simulink model "drone_position_control_sta_z_tuned"  (R2022a)
settings: Solver=ode4  StartTime=0.0  StopTime=42  FixedStep=.001  RelTol=1e-3
model workspace (MAT data in the model file):
  AttDyna_Ixx = 0.0211
  AttDyna_Iyy = 0.0219
  AttDyna_Izz = 0.0366
  AttDyna_JRP = 0.0001287
  ConEfficiency_drone_R = 0.225
  ConEfficiency_drone_cM = 1.779e-07
  ConEfficiency_drone_cT = 1.105e-05
  HeightNominalPlant = [1.4 9.8 1.105e-05 1148 -141.4]
  HeightSTAParams = [20 12 0.01 -22 8 8 0.005 3 5]
  PosDyna_GravityAcc = 9.8
  PosDyna_Mass = 1.4
  PowerUnit_CR = 1148
  PowerUnit_Tm = 0.02
  PowerUnit_wb = -141.4
undefined symbols (not defined in the file): earthRadius, Receive, Send
libraries: aerolibfltsims x3, slpidlib x3, aerolibanimutils x1
Description:
  | 高度专用离散 STA：加速度形式、限速前馈、倾斜重力补偿、条件积分。电机 PWM 共用 1000–2000 限幅。标称参数与实际物理参数分开。
settings Model: Creator=ZhangZheng  LastModifiedBy=13501
settings SolverCC: AlgebraicLoopSolver=TrustRegion
settings DataIOCC: ReturnWorkspaceOutputs=off
settings DebuggingCC: UnconnectedInputMsg=warning  UnconnectedOutputMsg=warning  UnconnectedLineMsg=warning  SFMachineParentedDataDiag=warning  ArithmeticOperatorsInVariantConditions=warning
settings SFSimCC: SimUseLocalCustomCode=off  CustomCodeUndefinedFunction=UseInterfaceOnly
settings RTWCC: RTWUseLocalCustomCode=off

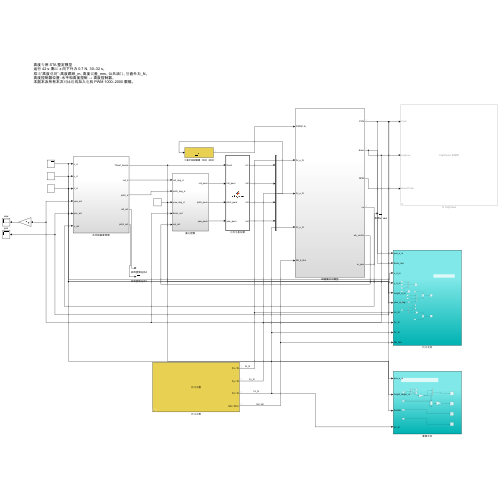
[thumbnail: Simulink's stored preview of the top-level diagram]
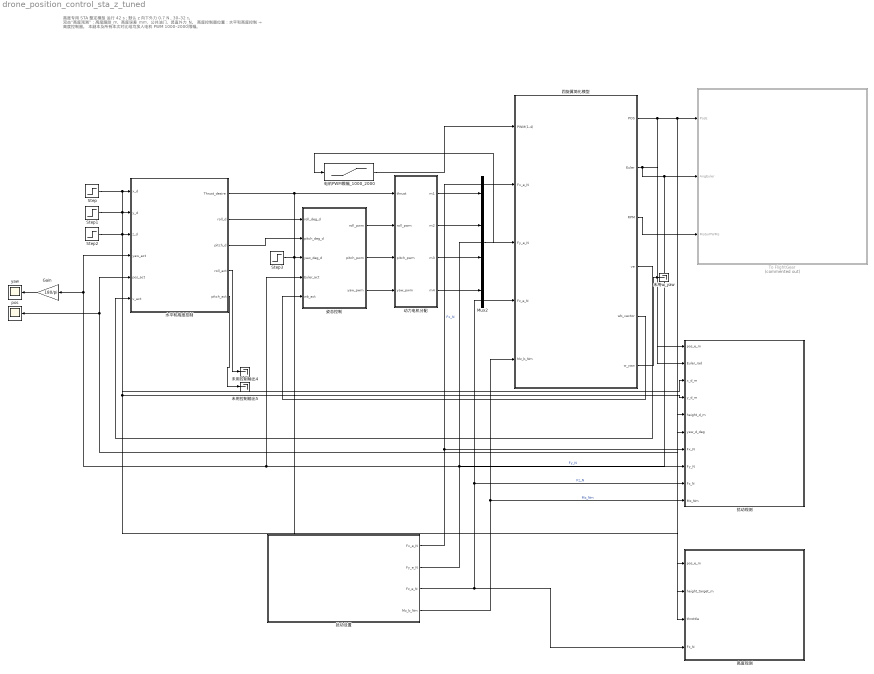
== system drone_position_control_sta_z_tuned ==
  note: 高度专用 STA 整定模型
      | 运行 42 s；默认 z 向下外力 0.7 N，30–32 s。
      | 双击“高度观测”：高度跟踪_m、高度误差_mm、公共油门、竖直外力_N。
      | 高度控制器位置：水平和高度控制 → 高度控制器。
      | 本副本及所有本次对比组均加入电机 PWM 1000–2000 限幅。
  Gain : Gain  Gain=180/pi
  Mux2 : Mux
  Step : Step  Time=5  After=5  SampleTime=0
  Step1 : Step  Time=10  After=5  SampleTime=0
  Step2 : Step  Time=0  After=10  SampleTime=0
  Step3 : Step  Time=15  After=5  SampleTime=0
  To FlightGear : Subsystem  Commented=on
      mask Display: disp('FlightGear 未启用')
  pos : Scope
  yaw : Scope
  动力电机分配 : MATLAB Function  TreatAsAtomicUnit=on
  四旋翼简化模型 : Subsystem
  姿态控制 : Subsystem
  扰动观测 : Subsystem
  扰动设置 : Subsystem  mask{Fx=0, Fy=0, Fz=0.7, Mz=0, t_on=30, t_off=32}
      mask prompts: Fx "x 向外力 Fx (N)"; Fy "y 向外力 Fy (N)"; Fz "z 向外力 Fz (N，向下为正)"; Mz "偏航力矩 Mz (N*m，绕机体 z 轴)"; t_on "施加时刻 (s)"; t_off "撤去时刻 (s)"
      mask help:
      | 默认：x 方向 0.7 N，30–32 s。其余通道为 0。
      | 单轴比较时只开启一个分量。y / z 测试使用 0.7 N，yaw 使用 0.02 N*m。
      | Fx、Fy、Fz 在惯性系表达；Mz 沿机体 z 轴。施加区间为 [施加时刻, 撤去时刻)。
      mask init:
      | validateattributes([Fx Fy Fz Mz],{'double'},{'real','finite','vector','numel',4});
      | validateattributes(t_on,{'double'},{'real','finite','scalar','nonnegative'});
      | validateattributes(t_off,{'double'},{'real','finite','scalar','>',t_on});
      mask Display:
      | disp('扰动设置');
      | port_label('output',1,'Fx / N');
      | port_label('output',2,'Fy / N');
      | port_label('output',3,'Fz / N');
      | port_label('output',4,'Mz / N*m');
  未用w_yaw : Terminator
  未用控制输出4 : Terminator
  未用控制输出5 : Terminator
  水平和高度控制 : Subsystem
  电机PWM限幅_1000_2000 : Saturate  UpperLimit=2000  LowerLimit=1000
  高度观测 : Subsystem
  wires:
  动力电机分配/4(m4) -> Mux2/4
  动力电机分配/3(m3) -> Mux2/3
  动力电机分配/2(m2) -> Mux2/2
  动力电机分配/1(m1) -> Mux2/1
  四旋翼简化模型/1(POS) -> 水平和高度控制/5(pos_act), pos/1, To FlightGear/1(PosE), 高度观测/1(pos_e_m), 扰动观测/1(pos_e_m)
  四旋翼简化模型/3(RPM) -> To FlightGear/3(MotorPWMs)
  姿态控制/1(roll_pwm) -> 动力电机分配/2(roll_pwm)
  姿态控制/2(pitch_pwm) -> 动力电机分配/3(pitch_pwm)
  姿态控制/3(yaw_pwm) -> 动力电机分配/4(yaw_pwm)
  四旋翼简化模型/5(wb_vector) -> 姿态控制/5(wb_act)
  四旋翼简化模型/2(Euler) -> 水平和高度控制/4(yaw_act), Gain/1, 姿态控制/4(Euler_act), To FlightGear/2(AngEuler), 扰动观测/2(Euler_rad)
  四旋翼简化模型/4(ve) -> 水平和高度控制/6(v_act)
  水平和高度控制/1(Thrust_desire) -> 动力电机分配/1(thrust), 高度观测/3(throttle)
  水平和高度控制/2(roll_d) -> 姿态控制/1(roll_deg_d)
  水平和高度控制/3(pitch_d) -> 姿态控制/2(pitch_deg_d)
  Step/1 -> 水平和高度控制/1(x_d), 扰动观测/3(x_d_m)
  Step1/1 -> 水平和高度控制/2(y_d), 扰动观测/4(y_d_m)
  Step2/1 -> 扰动观测/5(height_d_m), 高度观测/2(height_target_m), 水平和高度控制/3(z_d)
  Step3/1 -> 姿态控制/3(yaw_deg_d), 扰动观测/6(yaw_d_deg)
  Gain/1 -> yaw/1
  水平和高度控制/4(roll_act) -> 未用控制输出4/1
  水平和高度控制/5(pitch_act) -> 未用控制输出5/1
  四旋翼简化模型/6(w_yaw) -> 未用w_yaw/1
  扰动设置/1(Fx_e_N) -> 四旋翼简化模型/2(Fx_e_N), 扰动观测/7(Fx_N)  "Fx_N"
  扰动设置/2(Fy_e_N) -> 四旋翼简化模型/3(Fy_e_N), 扰动观测/8(Fy_N)  "Fy_N"
  扰动设置/3(Fz_e_N) -> 四旋翼简化模型/4(Fz_e_N), 扰动观测/9(Fz_N), 高度观测/4(Fz_N)  "Fz_N"
  扰动设置/4(Mz_b_Nm) -> 四旋翼简化模型/5(Mz_b_Nm), 扰动观测/10(Mz_Nm)  "Mz_Nm"
  Mux2/1 -> 电机PWM限幅_1000_2000/1
  电机PWM限幅_1000_2000/1 -> 四旋翼简化模型/1(PWM(1-4))

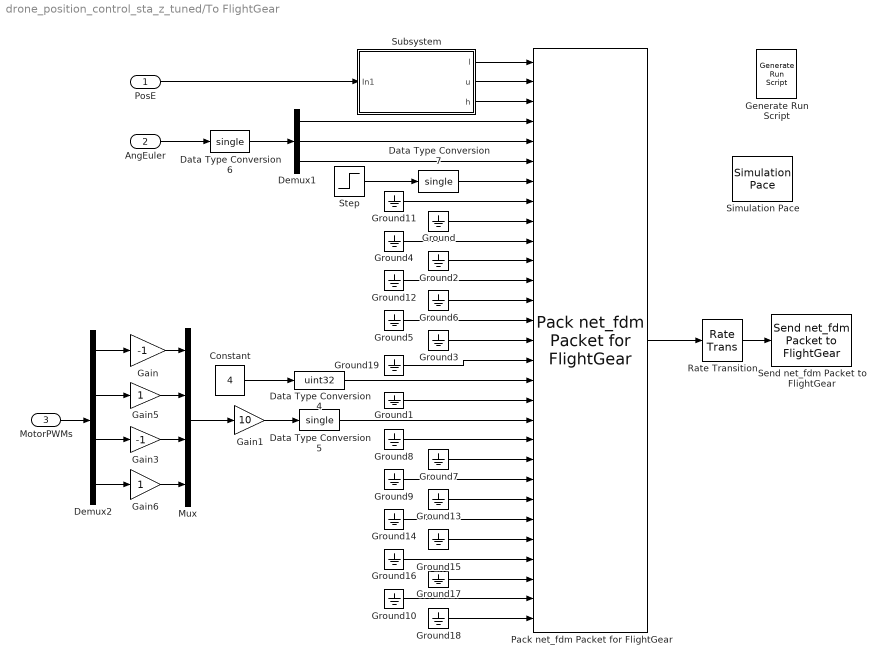
== system drone_position_control_sta_z_tuned/To FlightGear ==
  PosE : Inport
  AngEuler : Inport  Port=2
  MotorPWMs : Inport  Port=3
  Constant : Constant  Value=4
  Data Type Conversion4 : DataTypeConversion  OutDataTypeStr=uint32  SaturateOnIntegerOverflow=off  RndMeth=Floor
  Data Type Conversion5 : DataTypeConversion  OutDataTypeStr=single  SaturateOnIntegerOverflow=off  RndMeth=Floor
  Data Type Conversion6 : DataTypeConversion  OutDataTypeStr=single  SaturateOnIntegerOverflow=off  RndMeth=Floor
  Data Type Conversion7 : DataTypeConversion  OutDataTypeStr=single  SaturateOnIntegerOverflow=off  RndMeth=Floor
  Demux1 : Demux  Outputs=3
  Demux2 : Demux
  Gain : Gain  Gain=-1
  Gain1 : Gain  Gain=10
  Gain3 : Gain  Gain=-1
  Gain5 : Gain
  Gain6 : Gain
  Generate Run Script : aerolibfltsims/Generate Run Script  Architecture=Win64  dataFlow=Send-Receive  GeometryModelName=myownUAV  AirportId=KSFO  RunwayId=0  InitialAltitude=0  InitialHeading=0  OffsetDistance=0  OffsetAzimuth=0  InstallScenery=off  DisableShaders=off  OriginAddress=127.0.0.1  DestinationPort=5502  OriginPort=5505  LocalAddress=127.0.0.1  OutputFileName=runfg.bat  FlightGearBaseDirectory=E:\PX4PSP\FlightGear 2016.1.2
  Ground{,1..19} (20 alike) : Ground
  Mux : Mux
  Pack net_fdm Packet for FlightGear : aerolibfltsims/Pack net_fdm Packet for FlightGear  FlightGearVersion=v2016.1  ShowPositionAttitudeInputs=on  ShowVelocityAccelerationInputs=off  ShowControlSurfacePositionInputs=on  ShowEngineFuelInputs=on  ShowLandingGearInputs=off  ShowEnvironmentInputs=off  SampleTime=0.01  packetVersion=24
      settings: SourceProductBaseCode=AE
  Rate Transition : RateTransition
  Send net_fdm Packet to FlightGear : aerolibfltsims/Send net_fdm Packet to FlightGear  DestinationIpAddress=127.0.0.1  DestinationPort=5502  LocalIpPort=-1  varLen=off  SampleTime=0.005
      settings: SourceProductBaseCode=AE
  Simulation Pace : aerolibanimutils/Simulation Pace  SimulationPace=1  SleepMode=MATLAB Thread  OutputPaceError=off  SampleTime=-1
      settings: AttributesFormatString=%<SimulationPace> sec/sec
  Step : Step  Time=5  SampleTime=0
  Subsystem : Subsystem
  wires:
  Pack net_fdm Packet for FlightGear/1 -> Rate Transition/1
  Data Type Conversion7/1 -> Pack net_fdm Packet for FlightGear/7
  Ground8/1 -> Pack net_fdm Packet for FlightGear/20
  Ground/1 -> Pack net_fdm Packet for FlightGear/9
  Ground7/1 -> Pack net_fdm Packet for FlightGear/21
  Ground9/1 -> Pack net_fdm Packet for FlightGear/22
  Ground13/1 -> Pack net_fdm Packet for FlightGear/23
  Ground14/1 -> Pack net_fdm Packet for FlightGear/24
  Ground15/1 -> Pack net_fdm Packet for FlightGear/25
  Ground16/1 -> Pack net_fdm Packet for FlightGear/26
  Ground17/1 -> Pack net_fdm Packet for FlightGear/27
  Ground10/1 -> Pack net_fdm Packet for FlightGear/28
  Ground18/1 -> Pack net_fdm Packet for FlightGear/29
  Step/1 -> Data Type Conversion7/1
  Data Type Conversion4/1 -> Pack net_fdm Packet for FlightGear/17
  Ground1/1 -> Pack net_fdm Packet for FlightGear/18
  Ground3/1 -> Pack net_fdm Packet for FlightGear/15
  Ground5/1 -> Pack net_fdm Packet for FlightGear/14
  Ground6/1 -> Pack net_fdm Packet for FlightGear/13
  Ground4/1 -> Pack net_fdm Packet for FlightGear/10
  Ground11/1 -> Pack net_fdm Packet for FlightGear/8
  Constant/1 -> Data Type Conversion4/1
  Data Type Conversion5/1 -> Pack net_fdm Packet for FlightGear/19
  Ground2/1 -> Pack net_fdm Packet for FlightGear/11
  Ground12/1 -> Pack net_fdm Packet for FlightGear/12
  AngEuler/1 -> Data Type Conversion6/1
  MotorPWMs/1 -> Demux2/1
  Mux/1 -> Gain1/1
  Demux2/1 -> Gain/1
  Demux2/3 -> Gain3/1
  Gain/1 -> Mux/1
  Gain3/1 -> Mux/3
  Demux2/2 -> Gain5/1
  Gain5/1 -> Mux/2
  Demux2/4 -> Gain6/1
  Gain6/1 -> Mux/4
  Rate Transition/1 -> Send net_fdm Packet to FlightGear/1
  PosE/1 -> Subsystem/1(In1)
  Subsystem/1("l ") -> Pack net_fdm Packet for FlightGear/1
  Subsystem/2(u) -> Pack net_fdm Packet for FlightGear/2
  Subsystem/3(h) -> Pack net_fdm Packet for FlightGear/3
  Ground19/1 -> Pack net_fdm Packet for FlightGear/16
  Demux1/1 -> Pack net_fdm Packet for FlightGear/4
  Demux1/2 -> Pack net_fdm Packet for FlightGear/5
  Demux1/3 -> Pack net_fdm Packet for FlightGear/6
  Data Type Conversion6/1 -> Demux1/1
  Gain1/1 -> Data Type Conversion5/1

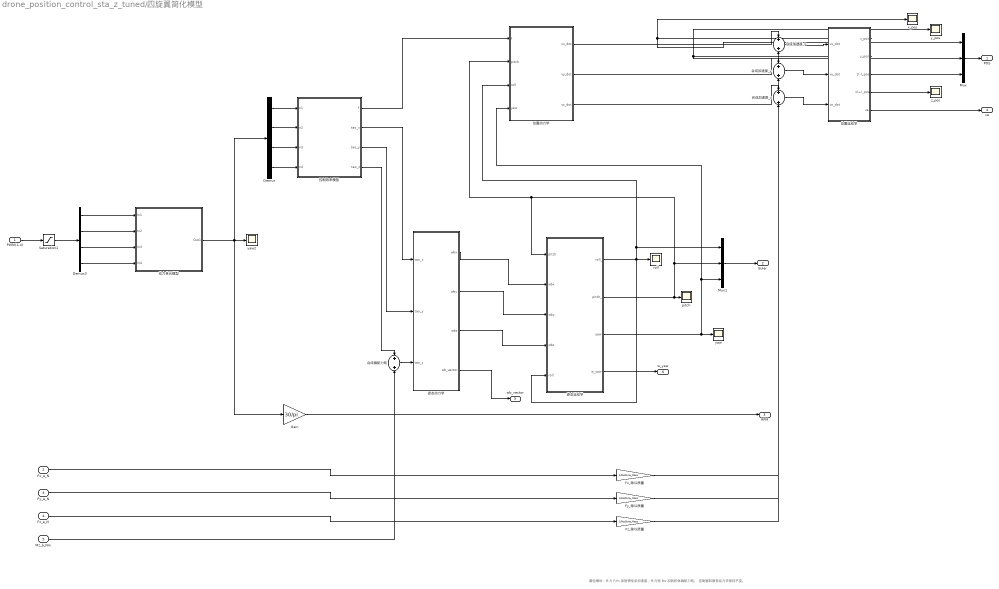
== system drone_position_control_sta_z_tuned/四旋翼简化模型 ==
  note: 黄色模块：外力 F/m 加到惯性系加速度；外力矩 Mz 加到机体偏航力矩。
      | 控制器和原有动力学保持不变。
  PWM(1-4) : Inport
  Fx_e_N : Inport  Port=2
  Fy_e_N : Inport  Port=3
  Fz_e_N : Inport  Port=4
  Mz_b_Nm : Inport  Port=5
  Demux : Demux
  Demux3 : Demux
  Fx_除以质量 : Gain  Gain=1/PosDyna_Mass
  Fy_除以质量 : Gain  Gain=1/PosDyna_Mass
  Fz_除以质量 : Gain  Gain=1/PosDyna_Mass
  Gain : Gain  Gain=30/pi
  Mux : Mux  Inputs=3
  Mux1 : Mux  Inputs=3
  Saturation1 : Saturate  UpperLimit=2000  LowerLimit=1000
  pitch : Scope
  roll : Scope
  x_pos : Scope
  y_pos : Scope
  yaw : Scope
  yaw2 : Scope
  z_pos : Scope
  位置动力学 : Subsystem
  位置运动学 : Subsystem
  动力单元模型 : Subsystem
  合成偏航力矩 : Sum
  合成加速度_x : Sum
  合成加速度_y : Sum
  合成加速度_z : Sum
  姿态动力学 : Subsystem
  姿态运动学 : Subsystem
  控制效率模型 : Subsystem
  POS : Outport  VectorParamsAs1DForOutWhenUnconnected=off
  Euler : Outport  Port=2  VectorParamsAs1DForOutWhenUnconnected=off
  RPM : Outport  Port=3  VectorParamsAs1DForOutWhenUnconnected=off
  ve : Outport  Port=4  VectorParamsAs1DForOutWhenUnconnected=off
  wb_vector : Outport  Port=5  VectorParamsAs1DForOutWhenUnconnected=off
  w_yaw : Outport  Port=6  VectorParamsAs1DForOutWhenUnconnected=off
  wires:
  Saturation1/1 -> Demux3/1
  姿态运动学/2(pitch_) -> 姿态运动学/1(pitch), 位置动力学/2(pitch), Mux1/2, pitch/1
  Demux/3 -> 控制效率模型/3(n3)
  PWM(1-4)/1 -> Saturation1/1
  Demux3/1 -> 动力单元模型/1(In1)
  Gain/1 -> RPM/1
  控制效率模型/3(tao_y) -> 姿态动力学/2(tao_y)
  Demux3/3 -> 动力单元模型/3(In3)
  Mux/1 -> POS/1
  Demux3/2 -> 动力单元模型/2(In2)
  Demux/2 -> 控制效率模型/2(n2)
  动力单元模型/1(Out1) -> Demux/1, yaw2/1, Gain/1
  Demux3/4 -> 动力单元模型/4(In4)
  Mux1/1 -> Euler/1
  控制效率模型/1(f) -> 位置动力学/1(f)
  Demux/4 -> 控制效率模型/4(n4)
  Demux/1 -> 控制效率模型/1(n1)
  控制效率模型/2(tao_x) -> 姿态动力学/1(tao_x)
  姿态动力学/1(wbx) -> 姿态运动学/2(wbx)
  姿态运动学/1(roll_) -> 姿态运动学/5(roll), roll/1, 位置动力学/3(roll), Mux1/1
  姿态动力学/4(wb_vector) -> wb_vector/1
  姿态运动学/3(yaw) -> 位置动力学/4(yaw), Mux1/3, yaw/1
  姿态动力学/3(wbz) -> 姿态运动学/4(wbz)
  姿态动力学/2(wby) -> 姿态运动学/3(wby)
  姿态运动学/4(w_yaw) -> w_yaw/1
  位置运动学/1(x_pos) -> x_pos/1, Mux/1
  位置运动学/2(y_pos) -> Mux/2, y_pos/1
  位置运动学/3(z(-)_pos) -> Mux/3
  位置运动学/4(z(+)_pos) -> z_pos/1
  位置运动学/5(ve) -> ve/1
  Fx_e_N/1 -> Fx_除以质量/1
  位置动力学/1(vx_dot) -> 合成加速度_x/1
  Fx_除以质量/1 -> 合成加速度_x/2
  合成加速度_x/1 -> 位置运动学/1(vx_dot)
  Fy_e_N/1 -> Fy_除以质量/1
  位置动力学/2(vy_dot) -> 合成加速度_y/1
  Fy_除以质量/1 -> 合成加速度_y/2
  合成加速度_y/1 -> 位置运动学/2(vy_dot)
  Fz_e_N/1 -> Fz_除以质量/1
  位置动力学/3(vz_dot) -> 合成加速度_z/1
  Fz_除以质量/1 -> 合成加速度_z/2
  合成加速度_z/1 -> 位置运动学/3(vz_dot)
  控制效率模型/4(tao_z) -> 合成偏航力矩/1
  Mz_b_Nm/1 -> 合成偏航力矩/2
  合成偏航力矩/1 -> 姿态动力学/3(tao_z)

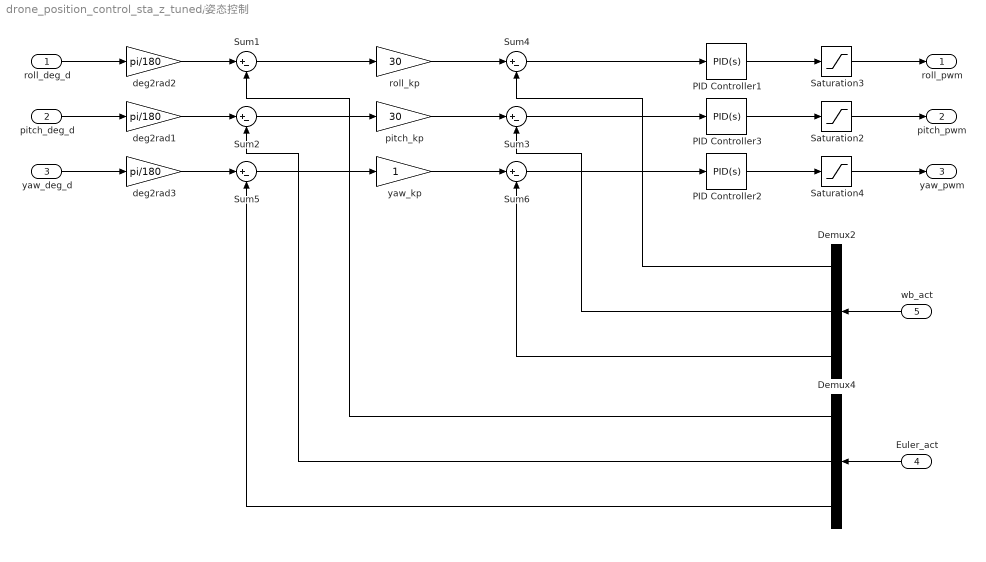
== system drone_position_control_sta_z_tuned/姿态控制 ==
  roll_deg_d : Inport
  pitch_deg_d : Inport  Port=2
  yaw_deg_d : Inport  Port=3
  Euler_act : Inport  Port=4
  wb_act : Inport  Port=5
  Demux2 : Demux  Outputs=3
  Demux4 : Demux  Outputs=3
  PID Controller1 : slpidlib/PID Controller  Controller=PID  Form=Parallel  TimeDomain=Continuous-time  UseExternalTs=off  SampleTime=-1  IntegratorMethod=Forward Euler  FilterMethod=Forward Euler  ControllerParametersSource=internal  P=0.3  I=1.4  UseKiTs=off  D=0.01  N=100  UseFilter=on  TunerSelectOption=Transfer Function Based (PID Tuner App)  InitialConditionSource=internal  InitialConditionForIntegrator=0  InitialConditionForFilter=0  DifferentiatorICPrevScaledInput=0  ExternalReset=none  TrackingMode=off  Kt=1  LimitOutput=off  SatLimitsSource=internal  UpperSaturationLimit=inf  LowerSaturationLimit=-inf  LinearizeAsGain=on  AntiWindupMode=none  Kb=1  POutMin=[]  POutMax=[]  IOutMin=[]  IOutMax=[]  DOutMin=[]  DOutMax=[]  NOutMin=[]  NOutMax=[]  SumOutMin=[]  SumOutMax=[]  SaturationOutMin=[]  SaturationOutMax=[]  PParamMin=[]  PParamMax=[]  IParamMin=[]  IParamMax=[]  DParamMin=[]  DParamMax=[]  NParamMin=[]  NParamMax=[]  KbParamMin=[]  KbParamMax=[]  KtParamMin=[]  KtParamMax=[]  KbOutMin=[]  KbOutMax=[]  KtOutMin=[]  KtOutMax=[]  IntegratorOutMin=[]  IntegratorOutMax=[]  FilterOutMin=[]  FilterOutMax=[]  SumI1OutMin=[]  SumI1OutMax=[]  SumI2OutMin=[]  SumI2OutMax=[]  SumI3OutMin=[]  SumI3OutMax=[]  SumI4OutMin=[]  SumI4OutMax=[]  SumDOutMin=[]  SumDOutMax=[]  DifferentiatorOutMin=[]  DifferentiatorOutMax=[]  FilterDiffOutCoefMin=[]  FilterDiffOutCoefMax=[]  ReciprocalOutMin=[]  ReciprocalOutMax=[]  SumDenOutMin=[]  SumDenOutMax=[]  SumNumOutMin=[]  SumNumOutMax=[]  DivideOutMin=[]  DivideOutMax=[]  UdiffTsProdOutMin=[]  UdiffTsProdOutMax=[]  NTsProdOutMin=[]  NTsProdOutMax=[]  UintegralTsProdOutMin=[]  UintegralTsProdOutMax=[]  UngainTsProdOutMin=[]  UngainTsProdOutMax=[]  IntegratorContinuousStateAttributes=''  IntegratorStateMustResolveToSignalObject=off  IntegratorRTWStateStorageClass=Auto  FilterContinuousStateAttributes=''  FilterStateMustResolveToSignalObject=off  FilterRTWStateStorageClass=Auto  ParallelPVariant=InternalParameters  IdealPVariant=Disabled  IVariant=InternalParameters  DVariant=InternalParameters  IntegratorVariant=Continuous  SatVariant=Disabled  AWVariant=Passthrough  PCopyVariant=Disabled  TRVariant=Disabled  FdbkBlocksVariant=Forward  IdealPFdbkVariant=Disabled  SatFdbkVariant=Disabled  DerivativeFilterVariant=ContFilter  NVariant=InternalParameters  NCopyVariant=Disabled  FilterICVariant=InternalICsFilter  IntegratorICVariant=InternalICs  ExternalResetVariant=Disabled  TRSumVariant=Passthrough  SumFdbkVariant=Disabled  SumVariant=Sum_PID  TsampFilterVariant=InternalTs  TsampNgainVariant=Passthrough  TsampIntegralVariant=Passthrough  ExternalSaturationOutDataTypeStr=Inherit: Same as second input  aMode=0
  PID Controller2 : slpidlib/PID Controller  Controller=PID  Form=Parallel  TimeDomain=Continuous-time  UseExternalTs=off  SampleTime=-1  IntegratorMethod=Forward Euler  FilterMethod=Forward Euler  ControllerParametersSource=internal  P=20  I=0  UseKiTs=off  D=0.1  N=100  UseFilter=on  TunerSelectOption=Transfer Function Based (PID Tuner App)  InitialConditionSource=internal  InitialConditionForIntegrator=0  InitialConditionForFilter=0  DifferentiatorICPrevScaledInput=0  ExternalReset=none  TrackingMode=off  Kt=1  LimitOutput=off  SatLimitsSource=internal  UpperSaturationLimit=inf  LowerSaturationLimit=-inf  LinearizeAsGain=on  AntiWindupMode=none  Kb=1  POutMin=[]  POutMax=[]  IOutMin=[]  IOutMax=[]  DOutMin=[]  DOutMax=[]  NOutMin=[]  NOutMax=[]  SumOutMin=[]  SumOutMax=[]  SaturationOutMin=[]  SaturationOutMax=[]  PParamMin=[]  PParamMax=[]  IParamMin=[]  IParamMax=[]  DParamMin=[]  DParamMax=[]  NParamMin=[]  NParamMax=[]  KbParamMin=[]  KbParamMax=[]  KtParamMin=[]  KtParamMax=[]  KbOutMin=[]  KbOutMax=[]  KtOutMin=[]  KtOutMax=[]  IntegratorOutMin=[]  IntegratorOutMax=[]  FilterOutMin=[]  FilterOutMax=[]  SumI1OutMin=[]  SumI1OutMax=[]  SumI2OutMin=[]  SumI2OutMax=[]  SumI3OutMin=[]  SumI3OutMax=[]  SumI4OutMin=[]  SumI4OutMax=[]  SumDOutMin=[]  SumDOutMax=[]  DifferentiatorOutMin=[]  DifferentiatorOutMax=[]  FilterDiffOutCoefMin=[]  FilterDiffOutCoefMax=[]  ReciprocalOutMin=[]  ReciprocalOutMax=[]  SumDenOutMin=[]  SumDenOutMax=[]  SumNumOutMin=[]  SumNumOutMax=[]  DivideOutMin=[]  DivideOutMax=[]  UdiffTsProdOutMin=[]  UdiffTsProdOutMax=[]  NTsProdOutMin=[]  NTsProdOutMax=[]  UintegralTsProdOutMin=[]  UintegralTsProdOutMax=[]  UngainTsProdOutMin=[]  UngainTsProdOutMax=[]  IntegratorContinuousStateAttributes=''  IntegratorStateMustResolveToSignalObject=off  IntegratorRTWStateStorageClass=Auto  FilterContinuousStateAttributes=''  FilterStateMustResolveToSignalObject=off  FilterRTWStateStorageClass=Auto  ParallelPVariant=InternalParameters  IdealPVariant=Disabled  IVariant=InternalParameters  DVariant=InternalParameters  IntegratorVariant=Continuous  SatVariant=Disabled  AWVariant=Passthrough  PCopyVariant=Disabled  TRVariant=Disabled  FdbkBlocksVariant=Forward  IdealPFdbkVariant=Disabled  SatFdbkVariant=Disabled  DerivativeFilterVariant=ContFilter  NVariant=InternalParameters  NCopyVariant=Disabled  FilterICVariant=InternalICsFilter  IntegratorICVariant=InternalICs  ExternalResetVariant=Disabled  TRSumVariant=Passthrough  SumFdbkVariant=Disabled  SumVariant=Sum_PID  TsampFilterVariant=InternalTs  TsampNgainVariant=Passthrough  TsampIntegralVariant=Passthrough  ExternalSaturationOutDataTypeStr=Inherit: Same as second input  aMode=0
  PID Controller3 : slpidlib/PID Controller  Controller=PID  Form=Parallel  TimeDomain=Continuous-time  UseExternalTs=off  SampleTime=-1  IntegratorMethod=Forward Euler  FilterMethod=Forward Euler  ControllerParametersSource=internal  P=0.3  I=1.4  UseKiTs=off  D=0.01  N=100  UseFilter=on  TunerSelectOption=Transfer Function Based (PID Tuner App)  InitialConditionSource=internal  InitialConditionForIntegrator=0  InitialConditionForFilter=0  DifferentiatorICPrevScaledInput=0  ExternalReset=none  TrackingMode=off  Kt=1  LimitOutput=off  SatLimitsSource=internal  UpperSaturationLimit=inf  LowerSaturationLimit=-inf  LinearizeAsGain=on  AntiWindupMode=none  Kb=1  POutMin=[]  POutMax=[]  IOutMin=[]  IOutMax=[]  DOutMin=[]  DOutMax=[]  NOutMin=[]  NOutMax=[]  SumOutMin=[]  SumOutMax=[]  SaturationOutMin=[]  SaturationOutMax=[]  PParamMin=[]  PParamMax=[]  IParamMin=[]  IParamMax=[]  DParamMin=[]  DParamMax=[]  NParamMin=[]  NParamMax=[]  KbParamMin=[]  KbParamMax=[]  KtParamMin=[]  KtParamMax=[]  KbOutMin=[]  KbOutMax=[]  KtOutMin=[]  KtOutMax=[]  IntegratorOutMin=[]  IntegratorOutMax=[]  FilterOutMin=[]  FilterOutMax=[]  SumI1OutMin=[]  SumI1OutMax=[]  SumI2OutMin=[]  SumI2OutMax=[]  SumI3OutMin=[]  SumI3OutMax=[]  SumI4OutMin=[]  SumI4OutMax=[]  SumDOutMin=[]  SumDOutMax=[]  DifferentiatorOutMin=[]  DifferentiatorOutMax=[]  FilterDiffOutCoefMin=[]  FilterDiffOutCoefMax=[]  ReciprocalOutMin=[]  ReciprocalOutMax=[]  SumDenOutMin=[]  SumDenOutMax=[]  SumNumOutMin=[]  SumNumOutMax=[]  DivideOutMin=[]  DivideOutMax=[]  UdiffTsProdOutMin=[]  UdiffTsProdOutMax=[]  NTsProdOutMin=[]  NTsProdOutMax=[]  UintegralTsProdOutMin=[]  UintegralTsProdOutMax=[]  UngainTsProdOutMin=[]  UngainTsProdOutMax=[]  IntegratorContinuousStateAttributes=''  IntegratorStateMustResolveToSignalObject=off  IntegratorRTWStateStorageClass=Auto  FilterContinuousStateAttributes=''  FilterStateMustResolveToSignalObject=off  FilterRTWStateStorageClass=Auto  ParallelPVariant=InternalParameters  IdealPVariant=Disabled  IVariant=InternalParameters  DVariant=InternalParameters  IntegratorVariant=Continuous  SatVariant=Disabled  AWVariant=Passthrough  PCopyVariant=Disabled  TRVariant=Disabled  FdbkBlocksVariant=Forward  IdealPFdbkVariant=Disabled  SatFdbkVariant=Disabled  DerivativeFilterVariant=ContFilter  NVariant=InternalParameters  NCopyVariant=Disabled  FilterICVariant=InternalICsFilter  IntegratorICVariant=InternalICs  ExternalResetVariant=Disabled  TRSumVariant=Passthrough  SumFdbkVariant=Disabled  SumVariant=Sum_PID  TsampFilterVariant=InternalTs  TsampNgainVariant=Passthrough  TsampIntegralVariant=Passthrough  ExternalSaturationOutDataTypeStr=Inherit: Same as second input  aMode=0
  Saturation2 : Saturate  UpperLimit=1  LowerLimit=-1
  Saturation3 : Saturate  UpperLimit=1  LowerLimit=-1
  Saturation4 : Saturate  UpperLimit=1  LowerLimit=-1
  Sum{1..6} (6 alike) : Sum  Inputs=|+-
  deg2rad1 : Gain  Gain=pi/180
  deg2rad2 : Gain  Gain=pi/180
  deg2rad3 : Gain  Gain=pi/180
  pitch_kp : Gain  Gain=30
  roll_kp : Gain  Gain=30
  yaw_kp : Gain
  roll_pwm : Outport  VectorParamsAs1DForOutWhenUnconnected=off
  pitch_pwm : Outport  Port=2  VectorParamsAs1DForOutWhenUnconnected=off
  yaw_pwm : Outport  Port=3  VectorParamsAs1DForOutWhenUnconnected=off
  wires:
  PID Controller1/1 -> Saturation3/1
  roll_deg_d/1 -> deg2rad2/1
  pitch_deg_d/1 -> deg2rad1/1
  Saturation2/1 -> pitch_pwm/1
  Sum2/1 -> pitch_kp/1
  Saturation3/1 -> roll_pwm/1
  PID Controller3/1 -> Saturation2/1
  deg2rad1/1 -> Sum2/1
  Sum1/1 -> roll_kp/1
  roll_kp/1 -> Sum4/1
  Saturation4/1 -> yaw_pwm/1
  yaw_kp/1 -> Sum6/1
  pitch_kp/1 -> Sum3/1
  deg2rad2/1 -> Sum1/1
  wb_act/1 -> Demux2/1
  PID Controller2/1 -> Saturation4/1
  yaw_deg_d/1 -> deg2rad3/1
  Demux2/3 -> Sum6/2
  deg2rad3/1 -> Sum5/1
  Demux2/2 -> Sum3/2
  Sum5/1 -> yaw_kp/1
  Demux4/3 -> Sum5/2
  Demux2/1 -> Sum4/2
  Demux4/2 -> Sum2/2
  Demux4/1 -> Sum1/2
  Euler_act/1 -> Demux4/1
  Sum4/1 -> PID Controller1/1
  Sum3/1 -> PID Controller3/1
  Sum6/1 -> PID Controller2/1

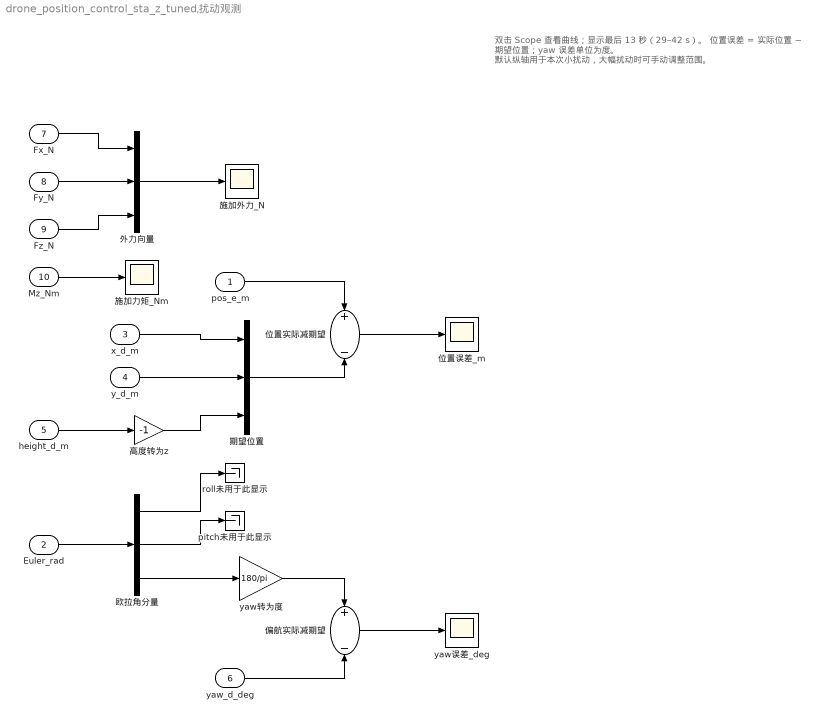
== system drone_position_control_sta_z_tuned/扰动观测 ==
  note: 双击 Scope 查看曲线；显示最后 13 秒（29–42 s）。
      | 位置误差 = 实际位置 − 期望位置；yaw 误差单位为度。
      | 默认纵轴用于本次小扰动，大幅扰动时可手动调整范围。
  pos_e_m : Inport
  Euler_rad : Inport  Port=2
  x_d_m : Inport  Port=3
  y_d_m : Inport  Port=4
  height_d_m : Inport  Port=5
  yaw_d_deg : Inport  Port=6
  Fx_N : Inport  Port=7
  Fy_N : Inport  Port=8
  Fz_N : Inport  Port=9
  Mz_Nm : Inport  Port=10
  pitch未用于此显示 : Terminator
  roll未用于此显示 : Terminator
  yaw误差_deg : Scope
  yaw转为度 : Gain  Gain=180/pi
  位置实际减期望 : Sum  Inputs=+-
  位置误差_m : Scope
  偏航实际减期望 : Sum  Inputs=+-
  外力向量 : Mux  Inputs=3
  施加力矩_Nm : Scope
  施加外力_N : Scope
  期望位置 : Mux  Inputs=3
  欧拉角分量 : Demux  Outputs=3
  高度转为z : Gain  Gain=-1
  wires:
  Mz_Nm/1 -> 施加力矩_Nm/1
  位置实际减期望/1 -> 位置误差_m/1
  高度转为z/1 -> 期望位置/3
  欧拉角分量/3 -> yaw转为度/1
  偏航实际减期望/1 -> yaw误差_deg/1
  外力向量/1 -> 施加外力_N/1
  Fx_N/1 -> 外力向量/1
  Fz_N/1 -> 外力向量/3
  yaw_d_deg/1 -> 偏航实际减期望/2
  Fy_N/1 -> 外力向量/2
  yaw转为度/1 -> 偏航实际减期望/1
  欧拉角分量/2 -> pitch未用于此显示/1
  欧拉角分量/1 -> roll未用于此显示/1
  Euler_rad/1 -> 欧拉角分量/1
  期望位置/1 -> 位置实际减期望/2
  pos_e_m/1 -> 位置实际减期望/1
  height_d_m/1 -> 高度转为z/1
  y_d_m/1 -> 期望位置/2
  x_d_m/1 -> 期望位置/1

== system drone_position_control_sta_z_tuned/扰动设置 ==
  Fx : Gain  Gain=Fx
  Fy : Gain  Gain=Fy
  Fz : Gain  Gain=Fz
  Mz : Gain  Gain=Mz
  持续时间窗口 : Sum
  撤去 : Step  Time=t_off  After=-1  SampleTime=0
  施加 : Step  Time=t_on  SampleTime=0
  Fx_e_N : Outport
  Fy_e_N : Outport  Port=2
  Fz_e_N : Outport  Port=3
  Mz_b_Nm : Outport  Port=4
  wires:
  施加/1 -> 持续时间窗口/1
  撤去/1 -> 持续时间窗口/2
  持续时间窗口/1 -> Fx/1, Fy/1, Fz/1, Mz/1
  Fx/1 -> Fx_e_N/1
  Fy/1 -> Fy_e_N/1
  Fz/1 -> Fz_e_N/1
  Mz/1 -> Mz_b_Nm/1

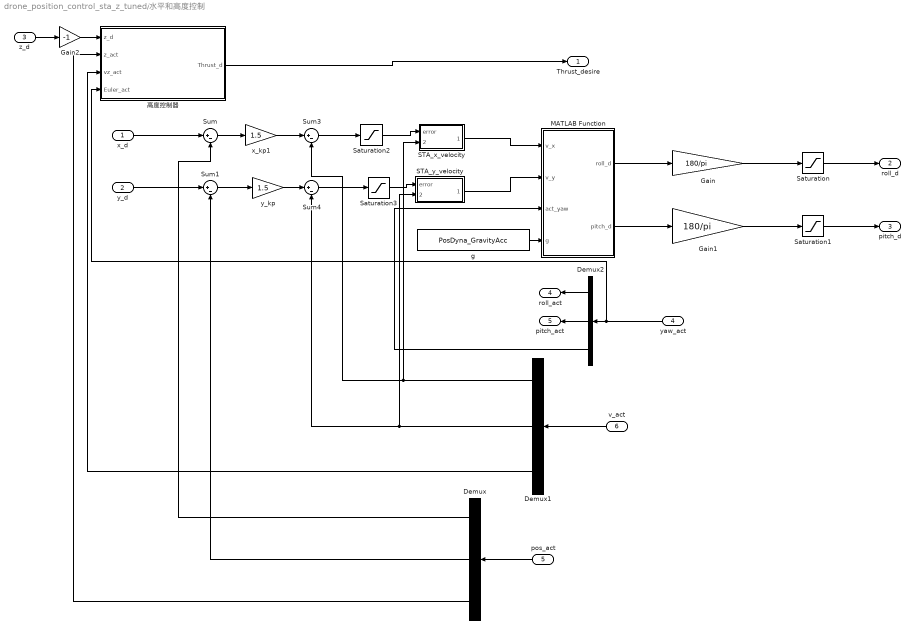
== system drone_position_control_sta_z_tuned/水平和高度控制 ==
  x_d : Inport
  y_d : Inport  Port=2
  z_d : Inport  Port=3
  yaw_act : Inport  Port=4
  pos_act : Inport  Port=5
  v_act : Inport  Port=6
  Demux : Demux  Outputs=3
  Demux1 : Demux  Outputs=3
  Demux2 : Demux  Outputs=3
  Gain : Gain  Gain=180/pi
  Gain1 : Gain  Gain=180/pi
  Gain2 : Gain  Gain=-1
  MATLAB Function : MATLAB Function  TreatAsAtomicUnit=on
  STA_x_velocity : Subsystem  Tag=STA:x_velocity  Description=水平 STA 试验：速度前馈 -lambda*v_actual；条件积分抗饱和；Ts=0.005s。源码 sta_velocity_ff_conditional.m 为说明副本，仿真运行模型内嵌函数。
  STA_y_velocity : Subsystem  Tag=STA:y_velocity  Description=水平 STA 试验：速度前馈 -lambda*v_actual；条件积分抗饱和；Ts=0.005s。源码 sta_velocity_ff_conditional.m 为说明副本，仿真运行模型内嵌函数。
  Saturation : Saturate  UpperLimit=10  LowerLimit=-20
  Saturation1 : Saturate  UpperLimit=10  LowerLimit=-10
  Saturation2 : Saturate  Description=保留完整速度误差；加速度指令在 STA 函数内限幅至正负 1.7 m/s^2。  UpperLimit=inf  LowerLimit=-inf
  Saturation3 : Saturate  Description=保留完整速度误差；加速度指令在 STA 函数内限幅至正负 1.7 m/s^2。  UpperLimit=inf  LowerLimit=-inf
  Sum{,1,3..4} (4 alike) : Sum  Inputs=|+-
  g : Constant  Value=PosDyna_GravityAcc
  x_kp1 : Gain  Gain=1.5
  y_kp : Gain  Gain=1.5
  高度控制器 : Subsystem  Description=高度专用 STA：NED z 向下，加速度单位控制律、限速前馈、倾斜重力补偿、条件积分。参数在模型工作区 HeightSTAParams。
  Thrust_desire : Outport  VectorParamsAs1DForOutWhenUnconnected=off
  roll_d : Outport  Port=2  VectorParamsAs1DForOutWhenUnconnected=off
  pitch_d : Outport  Port=3  VectorParamsAs1DForOutWhenUnconnected=off
  roll_act : Outport  Port=4  VectorParamsAs1DForOutWhenUnconnected=off
  pitch_act : Outport  Port=5  VectorParamsAs1DForOutWhenUnconnected=off
  wires:
  Saturation2/1 -> STA_x_velocity/1(error)
  Demux2/3 -> MATLAB Function/3(act_yaw)
  Demux2/1 -> roll_act/1
  yaw_act/1 -> Demux2/1, 高度控制器/4(Euler_act)
  Demux2/2 -> pitch_act/1
  pos_act/1 -> Demux/1
  Demux/2 -> Sum1/2
  Sum1/1 -> y_kp/1
  Sum4/1 -> Saturation3/1
  y_kp/1 -> Sum4/1
  y_d/1 -> Sum1/1
  Demux/1 -> Sum/2
  z_d/1 -> Gain2/1
  g/1 -> MATLAB Function/4(g)
  v_act/1 -> Demux1/1
  Saturation/1 -> roll_d/1
  Demux1/1 -> Sum3/2, STA_x_velocity/2(actual_velocity)
  MATLAB Function/2(pitch_d) -> Gain1/1
  Saturation1/1 -> pitch_d/1
  STA_x_velocity/1(control) -> MATLAB Function/1(v_x)
  Gain/1 -> Saturation/1
  MATLAB Function/1(roll_d) -> Gain/1
  Sum3/1 -> Saturation2/1
  STA_y_velocity/1(control) -> MATLAB Function/2(v_y)
  Demux1/2 -> Sum4/2, STA_y_velocity/2(actual_velocity)
  Saturation3/1 -> STA_y_velocity/1(error)
  x_kp1/1 -> Sum3/1
  x_d/1 -> Sum/1
  Gain1/1 -> Saturation1/1
  Sum/1 -> x_kp1/1
  高度控制器/1(Thrust_d) -> Thrust_desire/1
  Gain2/1 -> 高度控制器/1(z_d)
  Demux/3 -> 高度控制器/2(z_act)
  Demux1/3 -> 高度控制器/3(vz_act)

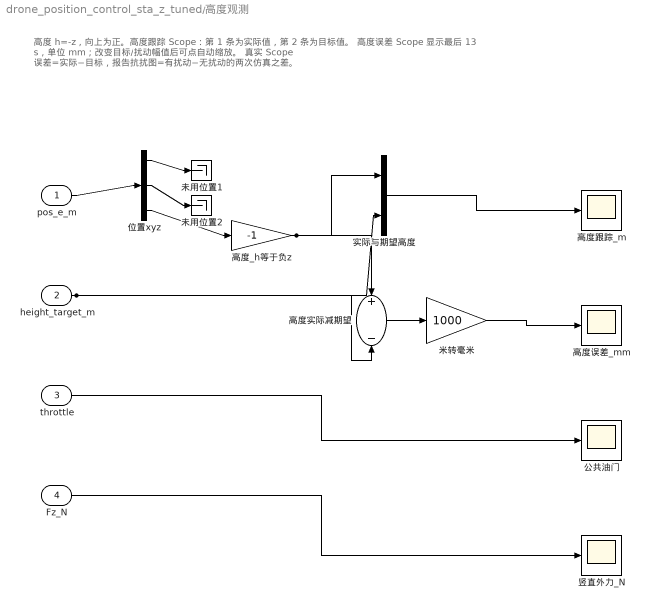
== system drone_position_control_sta_z_tuned/高度观测 ==
  note: 高度 h=-z，向上为正。高度跟踪 Scope：第 1 条为实际值，第 2 条为目标值。
      | 高度误差 Scope 显示最后 13 s，单位 mm；改变目标/扰动幅值后可点自动缩放。
      | 真实 Scope 误差=实际−目标，报告抗扰图=有扰动−无扰动的两次仿真之差。
  pos_e_m : Inport
  height_target_m : Inport  Port=2
  throttle : Inport  Port=3
  Fz_N : Inport  Port=4
  位置xyz : Demux  Outputs=3
  公共油门 : Scope
  实际与期望高度 : Mux  Inputs=2
  未用位置1 : Terminator
  未用位置2 : Terminator
  竖直外力_N : Scope
  米转毫米 : Gain  Gain=1000
  高度_h等于负z : Gain  Gain=-1
  高度实际减期望 : Sum  Inputs=+-
  高度误差_mm : Scope
  高度跟踪_m : Scope
  wires:
  pos_e_m/1 -> 位置xyz/1
  位置xyz/1 -> 未用位置1/1
  位置xyz/2 -> 未用位置2/1
  位置xyz/3 -> 高度_h等于负z/1
  高度_h等于负z/1 -> 实际与期望高度/1, 高度实际减期望/1
  height_target_m/1 -> 实际与期望高度/2, 高度实际减期望/2
  高度实际减期望/1 -> 米转毫米/1
  实际与期望高度/1 -> 高度跟踪_m/1
  米转毫米/1 -> 高度误差_mm/1
  throttle/1 -> 公共油门/1
  Fz_N/1 -> 竖直外力_N/1

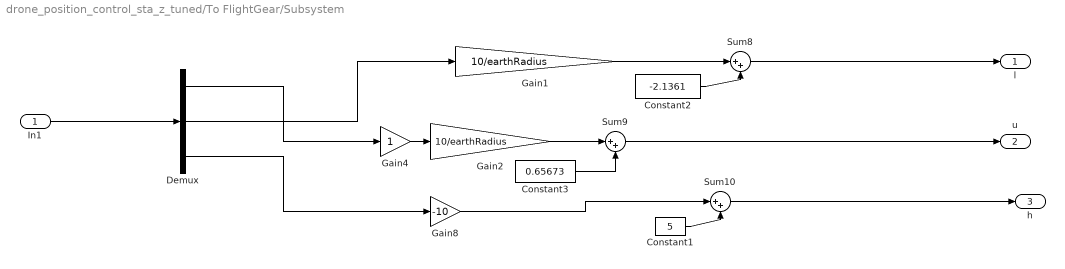
== system drone_position_control_sta_z_tuned/To FlightGear/Subsystem ==
  In1 : Inport
  Constant1 : Constant  Value=5  VectorParams1D=off
  Constant2 : Constant  Value=-2.1361  VectorParams1D=off
  Constant3 : Constant  Value=0.65673  VectorParams1D=off
  Demux : Demux  Outputs=3
  Gain1 : Gain  Gain=10/earthRadius
  Gain2 : Gain  Gain=10/earthRadius
  Gain4 : Gain
  Gain8 : Gain  Gain=-10
  Sum10 : Sum  Inputs=|++
  Sum8 : Sum  Inputs=|++
  Sum9 : Sum  Inputs=|++
  "l " : Outport  VectorParamsAs1DForOutWhenUnconnected=off
  u : Outport  Port=2  VectorParamsAs1DForOutWhenUnconnected=off
  h : Outport  Port=3  VectorParamsAs1DForOutWhenUnconnected=off
  wires:
  Constant3/1 -> Sum9/2
  Constant1/1 -> Sum10/2
  Demux/1 -> Gain4/1
  Demux/3 -> Gain8/1
  Constant2/1 -> Sum8/2
  Gain2/1 -> Sum9/1
  Gain1/1 -> Sum8/1
  Gain8/1 -> Sum10/1
  Demux/2 -> Gain1/1
  Gain4/1 -> Gain2/1
  Sum10/1 -> h/1
  Sum9/1 -> u/1
  In1/1 -> Demux/1
  Sum8/1 -> "l "/1

== system drone_position_control_sta_z_tuned/四旋翼简化模型/位置动力学 ==
  f : Inport
  pitch : Inport  Port=2
  roll : Inport  Port=3
  yaw : Inport  Port=4
  Constant : Constant  Value=PosDyna_Mass
  Constant3 : Constant  Value=PosDyna_GravityAcc
  pos_dyna : MATLAB Function  TreatAsAtomicUnit=on
  vx_dot : Outport  VectorParamsAs1DForOutWhenUnconnected=off
  vy_dot : Outport  Port=2  VectorParamsAs1DForOutWhenUnconnected=off
  vz_dot : Outport  Port=3  VectorParamsAs1DForOutWhenUnconnected=off
  wires:
  pos_dyna/1(vx_dot) -> vx_dot/1
  Constant/1 -> pos_dyna/2(m)
  pos_dyna/3(vz_dot) -> vz_dot/1
  pos_dyna/2(vy_dot) -> vy_dot/1
  Constant3/1 -> pos_dyna/3(g)
  yaw/1 -> pos_dyna/4(yaw)
  pitch/1 -> pos_dyna/5(pitch)
  roll/1 -> pos_dyna/6(roll)
  f/1 -> pos_dyna/1(f)

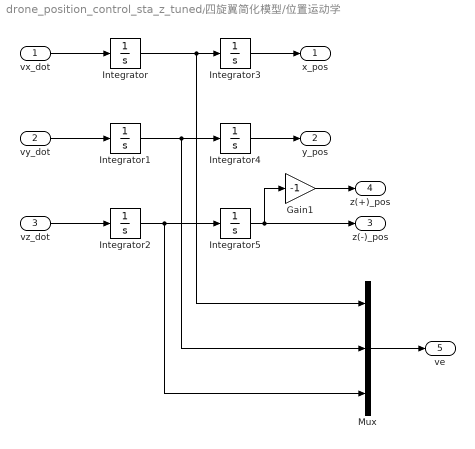
== system drone_position_control_sta_z_tuned/四旋翼简化模型/位置运动学 ==
  vx_dot : Inport
  vy_dot : Inport  Port=2
  vz_dot : Inport  Port=3
  Gain1 : Gain  Gain=-1
  Integrator{,1..5} (6 alike) : Integrator
  Mux : Mux  Inputs=3
  x_pos : Outport  VectorParamsAs1DForOutWhenUnconnected=off
  y_pos : Outport  Port=2  VectorParamsAs1DForOutWhenUnconnected=off
  z(-)_pos : Outport  Port=3  VectorParamsAs1DForOutWhenUnconnected=off
  z(+)_pos : Outport  Port=4  VectorParamsAs1DForOutWhenUnconnected=off
  ve : Outport  Port=5  VectorParamsAs1DForOutWhenUnconnected=off
  wires:
  Integrator1/1 -> Mux/2, Integrator4/1
  Integrator2/1 -> Mux/3, Integrator5/1
  Integrator5/1 -> z(-)_pos/1, Gain1/1
  vx_dot/1 -> Integrator/1
  Integrator4/1 -> y_pos/1
  Gain1/1 -> z(+)_pos/1
  vy_dot/1 -> Integrator1/1
  vz_dot/1 -> Integrator2/1
  Integrator/1 -> Mux/1, Integrator3/1
  Integrator3/1 -> x_pos/1
  Mux/1 -> ve/1

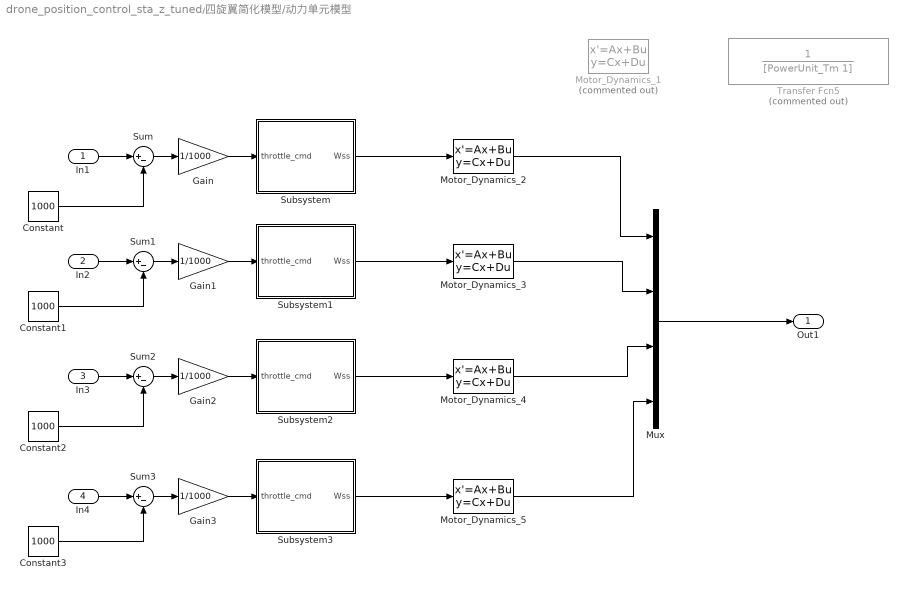
== system drone_position_control_sta_z_tuned/四旋翼简化模型/动力单元模型 ==
  In1 : Inport
  In2 : Inport  Port=2
  In3 : Inport  Port=3
  In4 : Inport  Port=4
  Constant{,1..3} (4 alike) : Constant  Value=1000
  Gain{,1..3} (4 alike) : Gain  Gain=1/1000
  Motor_Dynamics_1 : StateSpace  Commented=on  A=-1/PowerUnit_Tm  C=1/PowerUnit_Tm  D=0  InitialCondition=557.142*PowerUnit_Tm
  Motor_Dynamics_{2..5} (4 alike) : StateSpace  A=-1/PowerUnit_Tm  C=1/PowerUnit_Tm  D=0  InitialCondition=557.142*PowerUnit_Tm
  Mux : Mux
  Subsystem : Subsystem
  Subsystem1 : Subsystem
  Subsystem2 : Subsystem
  Subsystem3 : Subsystem
  Sum{,1..3} (4 alike) : Sum  Inputs=|+-
  Transfer Fcn5 : TransferFcn  Commented=on  Denominator=[PowerUnit_Tm 1]
  Out1 : Outport  VectorParamsAs1DForOutWhenUnconnected=off
  wires:
  Subsystem2/1(Wss) -> Motor_Dynamics_4/1
  Mux/1 -> Out1/1
  Subsystem1/1(Wss) -> Motor_Dynamics_3/1
  Subsystem3/1(Wss) -> Motor_Dynamics_5/1
  Motor_Dynamics_2/1 -> Mux/1
  Motor_Dynamics_4/1 -> Mux/3
  Subsystem/1(Wss) -> Motor_Dynamics_2/1
  Motor_Dynamics_3/1 -> Mux/2
  Motor_Dynamics_5/1 -> Mux/4
  In1/1 -> Sum/1
  Sum/1 -> Gain/1
  Gain/1 -> Subsystem/1("throttle_cmd ")
  Constant/1 -> Sum/2
  Constant1/1 -> Sum1/2
  Sum1/1 -> Gain1/1
  In2/1 -> Sum1/1
  Gain1/1 -> Subsystem1/1("throttle_cmd ")
  In3/1 -> Sum2/1
  Sum2/1 -> Gain2/1
  Constant2/1 -> Sum2/2
  Gain2/1 -> Subsystem2/1("throttle_cmd ")
  Constant3/1 -> Sum3/2
  Sum3/1 -> Gain3/1
  In4/1 -> Sum3/1
  Gain3/1 -> Subsystem3/1("throttle_cmd ")

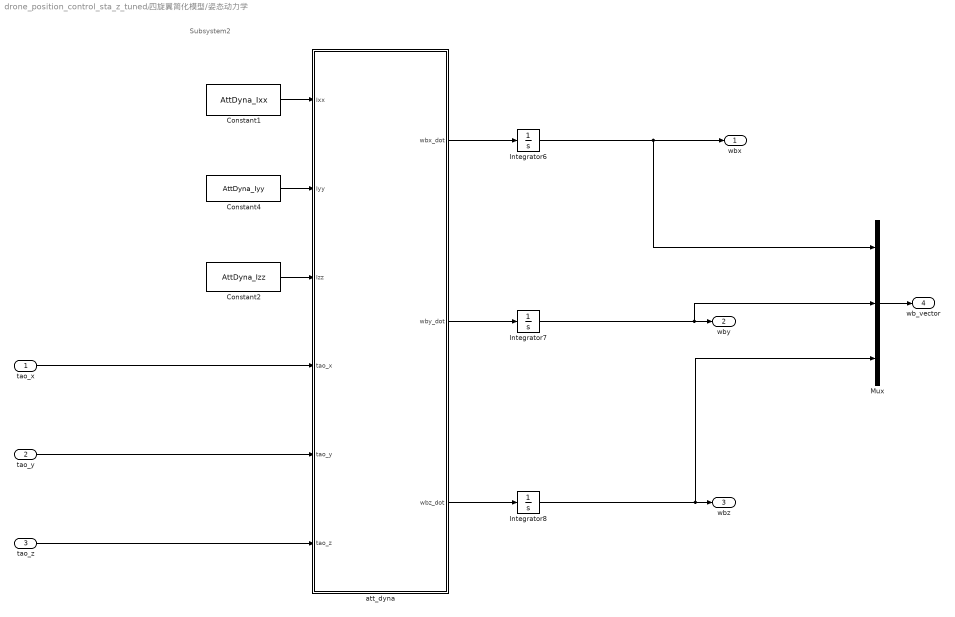
== system drone_position_control_sta_z_tuned/四旋翼简化模型/姿态动力学 ==
  note: Subsystem2
  tao_x : Inport
  tao_y : Inport  Port=2
  tao_z : Inport  Port=3
  Constant1 : Constant  Value=AttDyna_Ixx
  Constant2 : Constant  Value=AttDyna_Izz
  Constant4 : Constant  Value=AttDyna_Iyy
  Integrator6 : Integrator
  Integrator7 : Integrator
  Integrator8 : Integrator
  Mux : Mux  Inputs=3
  att_dyna : MATLAB Function  TreatAsAtomicUnit=on
  wbx : Outport  VectorParamsAs1DForOutWhenUnconnected=off
  wby : Outport  Port=2  VectorParamsAs1DForOutWhenUnconnected=off
  wbz : Outport  Port=3  VectorParamsAs1DForOutWhenUnconnected=off
  wb_vector : Outport  Port=4  VectorParamsAs1DForOutWhenUnconnected=off
  wires:
  att_dyna/3(wbz_dot) -> Integrator8/1
  att_dyna/2(wby_dot) -> Integrator7/1
  att_dyna/1(wbx_dot) -> Integrator6/1
  tao_y/1 -> att_dyna/5(tao_y)
  tao_z/1 -> att_dyna/6(tao_z)
  tao_x/1 -> att_dyna/4(tao_x)
  Integrator8/1 -> Mux/3, wbz/1
  Integrator6/1 -> Mux/1, wbx/1
  Integrator7/1 -> Mux/2, wby/1
  Constant2/1 -> att_dyna/3(Izz)
  Constant4/1 -> att_dyna/2(Iyy)
  Constant1/1 -> att_dyna/1(Ixx)
  Mux/1 -> wb_vector/1

== system drone_position_control_sta_z_tuned/四旋翼简化模型/姿态运动学 ==
  pitch : Inport
  wbx : Inport  Port=2
  wby : Inport  Port=3
  wbz : Inport  Port=4
  roll : Inport  Port=5
  Integrator10 : Integrator
  Integrator11 : Integrator
  Integrator9 : Integrator
  att_kine : MATLAB Function  TreatAsAtomicUnit=on
  roll_ : Outport  VectorParamsAs1DForOutWhenUnconnected=off
  pitch_ : Outport  Port=2  VectorParamsAs1DForOutWhenUnconnected=off
  yaw : Outport  Port=3  VectorParamsAs1DForOutWhenUnconnected=off
  w_yaw : Outport  Port=4  VectorParamsAs1DForOutWhenUnconnected=off
  wires:
  Integrator9/1 -> roll_/1
  att_kine/1(roll_dot) -> Integrator9/1
  att_kine/2(pitch_dot) -> Integrator10/1
  Integrator11/1 -> yaw/1
  Integrator10/1 -> pitch_/1
  att_kine/3(yaw_dot) -> w_yaw/1, Integrator11/1
  roll/1 -> att_kine/5(roll)
  pitch/1 -> att_kine/4(pitch)
  wbx/1 -> att_kine/1(wbx)
  wby/1 -> att_kine/2(wby)
  wbz/1 -> att_kine/3(wbz)

== system drone_position_control_sta_z_tuned/四旋翼简化模型/控制效率模型 ==
  n1 : Inport
  n2 : Inport  Port=2
  n3 : Inport  Port=3
  n4 : Inport  Port=4
  Constant5 : Constant  Value=ConEfficiency_drone_R
  Constant6 : Constant  Value=ConEfficiency_drone_cT
  Constant8 : Constant  Value=ConEfficiency_drone_cM
  control_efficiency : MATLAB Function  TreatAsAtomicUnit=on
  f : Outport  VectorParamsAs1DForOutWhenUnconnected=off
  tao_x : Outport  Port=2  VectorParamsAs1DForOutWhenUnconnected=off
  tao_y : Outport  Port=3  VectorParamsAs1DForOutWhenUnconnected=off
  tao_z : Outport  Port=4  VectorParamsAs1DForOutWhenUnconnected=off
  wires:
  control_efficiency/1(f) -> f/1
  control_efficiency/4(tao_z) -> tao_z/1
  n4/1 -> control_efficiency/4(n4)
  control_efficiency/2(tao_x) -> tao_x/1
  n3/1 -> control_efficiency/3(n3)
  control_efficiency/3(tao_y) -> tao_y/1
  n2/1 -> control_efficiency/2(n2)
  Constant8/1 -> control_efficiency/7(cm)
  n1/1 -> control_efficiency/1(n1)
  Constant5/1 -> control_efficiency/5(d)
  Constant6/1 -> control_efficiency/6(ct)

== system drone_position_control_sta_z_tuned/水平和高度控制/STA_x_velocity ==
  error : Inport
  actual_velocity : Inport  Port=2
  STA_formula : MATLAB Function  TreatAsAtomicUnit=on
  parameters : Constant  Description=仅此 XY 函数使用 [k1 k2 epsilon umin umax vmax Ts lambda]；lambda 必须和对应位置环增益一致。  Value=[3 1 .1 -1.7 1.7 1.7 .005 1.5]
  sample_error : ZeroOrderHold  SampleTime=0.0050000000000000001
  sample_velocity : ZeroOrderHold  SampleTime=.005
  v_state : UnitDelay  SampleTime=0.0050000000000000001  HasFrameUpgradeWarning=on
  control : Outport  VectorParamsAs1DForOutWhenUnconnected=off
  wires:
  error/1 -> sample_error/1
  sample_error/1 -> STA_formula/1(e)
  v_state/1 -> STA_formula/2(v)
  parameters/1 -> STA_formula/3(parameters)
  STA_formula/1(u) -> control/1
  STA_formula/2(v_next) -> v_state/1
  actual_velocity/1 -> sample_velocity/1
  sample_velocity/1 -> STA_formula/4(velocity)

== system drone_position_control_sta_z_tuned/水平和高度控制/STA_y_velocity ==
  error : Inport
  actual_velocity : Inport  Port=2
  STA_formula : MATLAB Function  TreatAsAtomicUnit=on
  parameters : Constant  Description=仅此 XY 函数使用 [k1 k2 epsilon umin umax vmax Ts lambda]；lambda 必须和对应位置环增益一致。  Value=[3 1 .1 -1.7 1.7 1.7 .005 1.5]
  sample_error : ZeroOrderHold  SampleTime=0.0050000000000000001
  sample_velocity : ZeroOrderHold  SampleTime=.005
  v_state : UnitDelay  SampleTime=0.0050000000000000001  HasFrameUpgradeWarning=on
  control : Outport  VectorParamsAs1DForOutWhenUnconnected=off
  wires:
  error/1 -> sample_error/1
  sample_error/1 -> STA_formula/1(e)
  v_state/1 -> STA_formula/2(v)
  parameters/1 -> STA_formula/3(parameters)
  STA_formula/1(u) -> control/1
  STA_formula/2(v_next) -> v_state/1
  actual_velocity/1 -> sample_velocity/1
  sample_velocity/1 -> STA_formula/4(velocity)

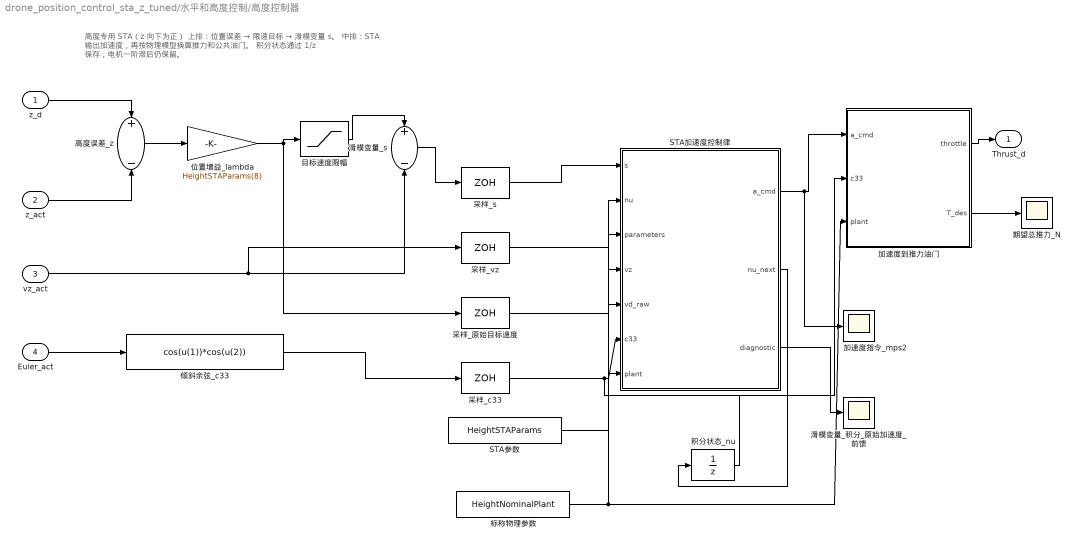
== system drone_position_control_sta_z_tuned/水平和高度控制/高度控制器 ==
  note: 高度专用 STA（z 向下为正）
      | 上排：位置误差 → 限速目标 → 滑模变量 s。
      | 中排：STA 输出加速度，再按物理模型换算推力和公共油门。
      | 积分状态通过 1/z 保存；电机一阶滞后仍保留。
  z_d : Inport
  z_act : Inport  Port=2
  vz_act : Inport  Port=3
  Euler_act : Inport  Port=4
  STA加速度控制律 : MATLAB Function  TreatAsAtomicUnit=on
  STA参数 : Constant  Value=HeightSTAParams
  位置增益_lambda : Gain  Gain=HeightSTAParams(8)
  倾斜余弦_c33 : Fcn  Expr=cos(u(1))*cos(u(2))
  加速度到推力油门 : MATLAB Function  TreatAsAtomicUnit=on
  加速度指令_mps2 : Scope
  期望总推力_N : Scope
  标称物理参数 : Constant  Value=HeightNominalPlant
  滑模变量_s : Sum  Inputs=+-
  滑模变量_积分_原始加速度_前馈 : Scope
  目标速度限幅 : Saturate  UpperLimit=HeightSTAParams(9)  LowerLimit=-HeightSTAParams(9)
  积分状态_nu : UnitDelay  SampleTime=.005  HasFrameUpgradeWarning=on
  采样_c33 : ZeroOrderHold  SampleTime=.005
  采样_s : ZeroOrderHold  SampleTime=.005
  采样_vz : ZeroOrderHold  SampleTime=.005
  采样_原始目标速度 : ZeroOrderHold  SampleTime=.005
  高度误差_z : Sum  Inputs=+-
  Thrust_d : Outport
  wires:
  z_d/1 -> 高度误差_z/1
  z_act/1 -> 高度误差_z/2
  高度误差_z/1 -> 位置增益_lambda/1
  位置增益_lambda/1 -> 目标速度限幅/1, 采样_原始目标速度/1
  目标速度限幅/1 -> 滑模变量_s/1
  vz_act/1 -> 滑模变量_s/2, 采样_vz/1
  Euler_act/1 -> 倾斜余弦_c33/1
  滑模变量_s/1 -> 采样_s/1
  倾斜余弦_c33/1 -> 采样_c33/1
  采样_s/1 -> STA加速度控制律/1(s)
  积分状态_nu/1 -> STA加速度控制律/2(nu)
  STA参数/1 -> STA加速度控制律/3(parameters)
  采样_vz/1 -> STA加速度控制律/4(vz)
  采样_原始目标速度/1 -> STA加速度控制律/5(vd_raw)
  采样_c33/1 -> STA加速度控制律/6(c33), 加速度到推力油门/2(c33)
  标称物理参数/1 -> STA加速度控制律/7(plant), 加速度到推力油门/3(plant)
  STA加速度控制律/2(nu_next) -> 积分状态_nu/1
  STA加速度控制律/1(a_cmd) -> 加速度到推力油门/1(a_cmd), 加速度指令_mps2/1
  加速度到推力油门/1(throttle) -> Thrust_d/1
  STA加速度控制律/3(diagnostic) -> 滑模变量_积分_原始加速度_前馈/1
  加速度到推力油门/2(T_des) -> 期望总推力_N/1

== system drone_position_control_sta_z_tuned/四旋翼简化模型/动力单元模型/Subsystem ==
  "throttle_cmd " : Inport
  CR : Gain  Gain=PowerUnit_CR
  Sum : Sum  Inputs=|++
  wb(转速常参数) : Constant  Value=PowerUnit_wb
  Wss : Outport  VectorParamsAs1DForOutWhenUnconnected=off
  wires:
  "throttle_cmd "/1 -> CR/1
  CR/1 -> Sum/1
  wb(转速常参数)/1 -> Sum/2
  Sum/1 -> Wss/1  "Wss"

== system drone_position_control_sta_z_tuned/四旋翼简化模型/动力单元模型/Subsystem1 ==
  "throttle_cmd " : Inport
  CR : Gain  Gain=PowerUnit_CR
  Sum : Sum  Inputs=|++
  wb(转速常参数) : Constant  Value=PowerUnit_wb
  Wss : Outport  VectorParamsAs1DForOutWhenUnconnected=off
  wires:
  Sum/1 -> Wss/1  "Wss"
  wb(转速常参数)/1 -> Sum/2
  CR/1 -> Sum/1
  "throttle_cmd "/1 -> CR/1

== system drone_position_control_sta_z_tuned/四旋翼简化模型/动力单元模型/Subsystem2 ==
  "throttle_cmd " : Inport
  CR : Gain  Gain=PowerUnit_CR
  Sum : Sum  Inputs=|++
  wb(转速常参数) : Constant  Value=PowerUnit_wb
  Wss : Outport  VectorParamsAs1DForOutWhenUnconnected=off
  wires:
  "throttle_cmd "/1 -> CR/1
  CR/1 -> Sum/1
  wb(转速常参数)/1 -> Sum/2
  Sum/1 -> Wss/1  "Wss"

== system drone_position_control_sta_z_tuned/四旋翼简化模型/动力单元模型/Subsystem3 ==
  "throttle_cmd " : Inport
  CR : Gain  Gain=PowerUnit_CR
  Sum : Sum  Inputs=|++
  wb(转速常参数) : Constant  Value=PowerUnit_wb
  Wss : Outport  VectorParamsAs1DForOutWhenUnconnected=off
  wires:
  Sum/1 -> Wss/1  "Wss"
  wb(转速常参数)/1 -> Sum/2
  CR/1 -> Sum/1
  "throttle_cmd "/1 -> CR/1

== matlab function drone_position_control_sta_z_tuned/水平和高度控制/高度控制器/STA加速度控制律 ==
  data: s input; a_cmd output; nu input; parameters input; vz input; vd_raw input; c33 input; plant input; nu_next output; diagnostic output
function [a_cmd, nu_next, diagnostic] = height_sta_acceleration(s, nu, parameters, vz, vd_raw, c33, plant)
%#codegen
% 高度专用离散 STA：输出惯性系 z 向加速度，向下为正。
% s = sat(lambda*(z_d-z), +/-vlim) - vz，单位 m/s。
% nu 是加速度单位的积分状态，不是飞机速度。
% parameters = [k1 k2 epsilon amin amax nu_max Ts lambda vlim]。
% plant = [m_nom g kf CR omega0]，控制器标称值与实际质量分开。
% 仅对分段恒定位置目标使用本前馈；阶跃瞬间不计算冲激导数。
k1=parameters(1); k2=parameters(2); epsilon=parameters(3);
amin=parameters(4); amax=parameters(5); nu_max=parameters(6);
Ts=parameters(7); lambda=parameters(8); vlim=parameters(9);
m=plant(1); g=plant(2); kf=plant(3); CR=plant(4); omega0=plant(5);

% 目标速度限幅时是常数，此时前馈必须为零。
a_ff=0;
if abs(vd_raw)<vlim
    a_ff=-lambda*vz;
end
sigma=min(max(s/epsilon,-1),1);
a_raw=a_ff+k1*sqrt(max(abs(s),epsilon))*sigma+nu;

% 同时考虑设计加速度限幅、最大油门和非负推力。
ctilt=min(max(c33,0.2),1);
Tmax=4*kf*(CR+omega0)^2;
lo=max(amin,g-Tmax*ctilt/m);
hi=min(amax,g);
a_cmd=min(max(a_raw,lo),hi);

% 条件积分：饱和且积分方向加重饱和时暂停；反向积分仍允许。
nu_dot=k2*sigma;
if (a_raw>hi && nu_dot>0)||(a_raw<lo && nu_dot<0)
    nu_dot=0;
end
nu_next=min(max(nu+Ts*nu_dot,-nu_max),nu_max);
diagnostic=[s;nu;a_raw;a_ff];
end

== matlab function drone_position_control_sta_z_tuned/水平和高度控制/高度控制器/加速度到推力油门 ==
  data: a_cmd input; throttle output; c33 input; plant input; T_des output
function [throttle, T_des] = height_acceleration_to_throttle(a_cmd,c33,plant)
%#codegen
% a_z=g-T*cos(phi)*cos(theta)/m；转为总推力，再转为公共油门。
% 此处使用稳态逆映射，原模型的 0.02 s 电机滞后仍然保留。
m=plant(1); g=plant(2); kf=plant(3); CR=plant(4); omega0=plant(5);
ctilt=min(max(c33,0.2),1);
T_des=max(0,m*(g-a_cmd)/ctilt);
omega_des=sqrt(T_des/(4*kf));
throttle=min(max((omega_des-omega0)/CR,0),1);
end

== matlab function drone_position_control_sta_z_tuned/水平和高度控制/STA_x_velocity/STA_formula ==
  data: e input; u output; v input; parameters input; v_next output; velocity input
function [u, v_next] = sta_velocity_ff_conditional(e, v, parameters, velocity)
%#codegen
% 水平速度环：带目标速度变化补偿、边界层和条件积分的离散 STA。
% e = v_desired - v_actual，velocity 是同一惯性系方向的实际速度。
% v 是控制器积分状态，不是飞机的实际速度。
% parameters = [k1 k2 epsilon umin umax vmax Ts lambda]。
% 本参数顺序仅用于此试验副本的 x/y 速度环；z 环沿用原有函数。
% 当位置目标在两次阶跃之间保持不变，v_desired=lambda*(pos_d-pos)，
% 因而 dot(v_desired)=-lambda*velocity。连续轨迹需要另行提供正确前馈。

k1 = parameters(1);
k2 = parameters(2);
epsilon = parameters(3);
umin = parameters(4);
umax = parameters(5);
vmax = parameters(6);
Ts = parameters(7);
lambda = parameters(8);

sigma = min(max(e / epsilon, -1), 1);
acceleration_ff = -lambda * velocity;
u_raw = acceleration_ff + k1 * sqrt(max(abs(e), epsilon)) * sigma + v;
u = min(max(u_raw, umin), umax);

% 条件积分：已饱和且积分还会加重饱和时，暂停积分。
% 若积分能够帮助退出饱和，则正常更新。
v_dot = k2 * sigma;
if (u_raw > umax && v_dot > 0) || (u_raw < umin && v_dot < 0)
    v_dot = 0;
end
v_next = min(max(v + Ts * v_dot, -vmax), vmax);
end

== matlab function drone_position_control_sta_z_tuned/水平和高度控制/STA_y_velocity/STA_formula ==
  data: e input; u output; v input; parameters input; v_next output; velocity input
function [u, v_next] = sta_velocity_ff_conditional(e, v, parameters, velocity)
%#codegen
% 水平速度环：带目标速度变化补偿、边界层和条件积分的离散 STA。
% e = v_desired - v_actual，velocity 是同一惯性系方向的实际速度。
% v 是控制器积分状态，不是飞机的实际速度。
% parameters = [k1 k2 epsilon umin umax vmax Ts lambda]。
% 本参数顺序仅用于此试验副本的 x/y 速度环；z 环沿用原有函数。
% 当位置目标在两次阶跃之间保持不变，v_desired=lambda*(pos_d-pos)，
% 因而 dot(v_desired)=-lambda*velocity。连续轨迹需要另行提供正确前馈。

k1 = parameters(1);
k2 = parameters(2);
epsilon = parameters(3);
umin = parameters(4);
umax = parameters(5);
vmax = parameters(6);
Ts = parameters(7);
lambda = parameters(8);

sigma = min(max(e / epsilon, -1), 1);
acceleration_ff = -lambda * velocity;
u_raw = acceleration_ff + k1 * sqrt(max(abs(e), epsilon)) * sigma + v;
u = min(max(u_raw, umin), umax);

% 条件积分：已饱和且积分还会加重饱和时，暂停积分。
% 若积分能够帮助退出饱和，则正常更新。
v_dot = k2 * sigma;
if (u_raw > umax && v_dot > 0) || (u_raw < umin && v_dot < 0)
    v_dot = 0;
end
v_next = min(max(v + Ts * v_dot, -vmax), vmax);
end

== matlab function drone_position_control_sta_z_tuned/四旋翼简化模型/姿态动力学/att_dyna ==
  data: Ixx input; Iyy input; Izz input; tao_x input; tao_y input; tao_z input; wbx_dot output; wby_dot output; wbz_dot output
function [wbx_dot,wby_dot,wbz_dot] = att_dyna(Ixx,Iyy,Izz,tao_x,tao_y,tao_z)
% wb = [wbx wby wbz]';
% wb_cha = [   0 -wbz   wby;
%            wbz    0  -wbx;
%           -wby  wbx     0];
% I = [Ixx   0   0;
%        0 Iyy   0;
%        0   0 Izz];
I_inv = [1/Ixx     0     0;
             0 1/Iyy     0;
             0     0 1/Izz];
tao = [tao_x tao_y tao_z]';
% G_x = Jrp * wby * (n1+n2-n3-n4);
% G_y = Jrp * wbx * (-n1-n2+n3+n4);
% G_z = 0;  
% G = [G_x G_y G_z]';
wb_dot = I_inv * (tao);
wbx_dot = wb_dot(1,1);
wby_dot = wb_dot(2,1);
wbz_dot = wb_dot(3,1);
end

== matlab function drone_position_control_sta_z_tuned/四旋翼简化模型/位置动力学/pos_dyna ==
  data: f input; vx_dot output; m input; g input; yaw input; pitch input; roll input; vy_dot output; vz_dot output
function [vx_dot,vy_dot,vz_dot] = pos_dyna(f,m,g,yaw,pitch,roll)
%位置动力学
%忽略了角速度和线速度的叉乘
vx_dot = (sin(roll)*sin(yaw) + cos(roll)*cos(yaw)*sin(pitch))*f/m;
vy_dot = (cos(roll)*sin(pitch)*sin(yaw) - cos(yaw)*sin(roll))*f/m;
vz_dot = (cos(pitch)*cos(roll)*f/m)+g;
end

== matlab function drone_position_control_sta_z_tuned/四旋翼简化模型/姿态运动学/att_kine ==
  data: wbx input; roll_dot output; wby input; wbz input; pitch input; pitch_dot output; yaw_dot output; roll input
function [roll_dot,pitch_dot,yaw_dot] = att_kine(wbx,wby,wbz,pitch,roll)
%姿态运动学
roll_dot = wbx + tan(pitch)*sin(roll)*wby + tan(pitch)*cos(roll)*wbz;
pitch_dot = cos(roll)*wby - sin(roll)*wbz;
yaw_dot = (sin(roll)/cos(pitch))*wby + (cos(roll)/cos(pitch))*wbz;
end

== matlab function drone_position_control_sta_z_tuned/四旋翼简化模型/控制效率模型/control_efficiency ==
  data: n1 input; f output; n2 input; n3 input; n4 input; tao_x output; tao_y output; tao_z output; d input; ct input; cm input
function [f,tao_x,tao_y,tao_z] = control_efficiency(n1,n2,n3,n4,d,ct,cm)
%控制效率模型
%X型机架
%3↓   1↑
%  \ /
%  / \
%2↑   4↓
%转速单位是弧度
f = -1*ct*(n1^2 + n2^2 + n3^2 + n4^2);%z轴朝下，所以拉力为负
tao_x = d*ct*sin(pi/4)*(-n1^2 + n2^2 + n3^2 - n4^2) / 2;
tao_y = d*ct*sin(pi/4)*(n1^2 - n2^2 + n3^2 - n4^2) / 2;
tao_z = cm*(n1^2 + n2^2 - n3^2 - n4^2);
%十字型
% f = ct*(n1^2 + n2^2 + n3^2 + n4^2);
% tao_x = -d*ct*n2^2 + d*ct*n4^2;
% tao_y =  d*ct*n1^2 - d*ct*n3^2;
% tao_z = cm*(n1^2 - n2^2 + n3^2 - n4^2);
end

== matlab function drone_position_control_sta_z_tuned/动力电机分配 ==
  data: thrust input; m1 output; m2 output; m3 output; m4 output; roll_pwm input; pitch_pwm input; yaw_pwm input
function [m1,m2,m3,m4] = motor_mixer(thrust,roll_pwm,pitch_pwm,yaw_pwm)
%输入的是都是占空比（0-1）之间
%输出四个电机的指令值，1000-2000
%这里采用x型机架，x型机架的分配和十字型的不一样

K = 1000;%将输入定在0-1000
pwm_base = 1000;%PWM从1000开始

m1 = (thrust - roll_pwm + pitch_pwm + yaw_pwm) * K + pwm_base;
m2 = (thrust + roll_pwm - pitch_pwm + yaw_pwm) * K + pwm_base;
m3 = (thrust + roll_pwm + pitch_pwm - yaw_pwm) * K + pwm_base;
m4 = (thrust - roll_pwm - pitch_pwm - yaw_pwm) * K + pwm_base;
end

== matlab function drone_position_control_sta_z_tuned/水平和高度控制/MATLAB Function ==
  data: v_x input; roll_d output; v_y input; act_yaw input; g input; pitch_d output
function [roll_d, pitch_d] = fcn(v_x,v_y,act_yaw,g)
%v_x,v_y是经过速度环pid控制之后的输出
%yaw是实际的yaw角度,单位是弧度制,并且matlab的三角函数接收的是弧度制
%g是重力加速度
%输出的角度也是弧度制
A_INV = [sin(act_yaw) -cos(act_yaw);
         cos(act_yaw)  sin(act_yaw)];
desire_roll_pitch = -1*(1/g) * A_INV * [v_x;v_y]; 
roll_d = desire_roll_pitch(1);
pitch_d = desire_roll_pitch(2);
